simulink model "FuzzyPID_modle"  (R2024b)
settings: Solver=ode4  StartTime=0.0  StopTime=100  FixedStep=0.5  RelTol=1e-3
undefined symbols (not defined in the file): DiscIntNeverNeededParam
libraries: fuzblock x2, slpidlib x1
settings Model: Creator=33242  LastModifiedBy=33242

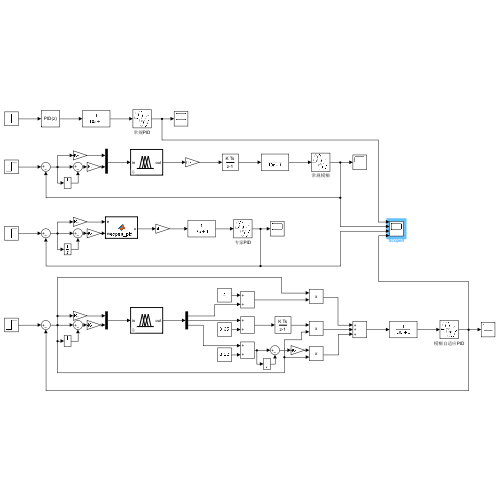
[thumbnail: Simulink's stored preview of the top-level diagram]
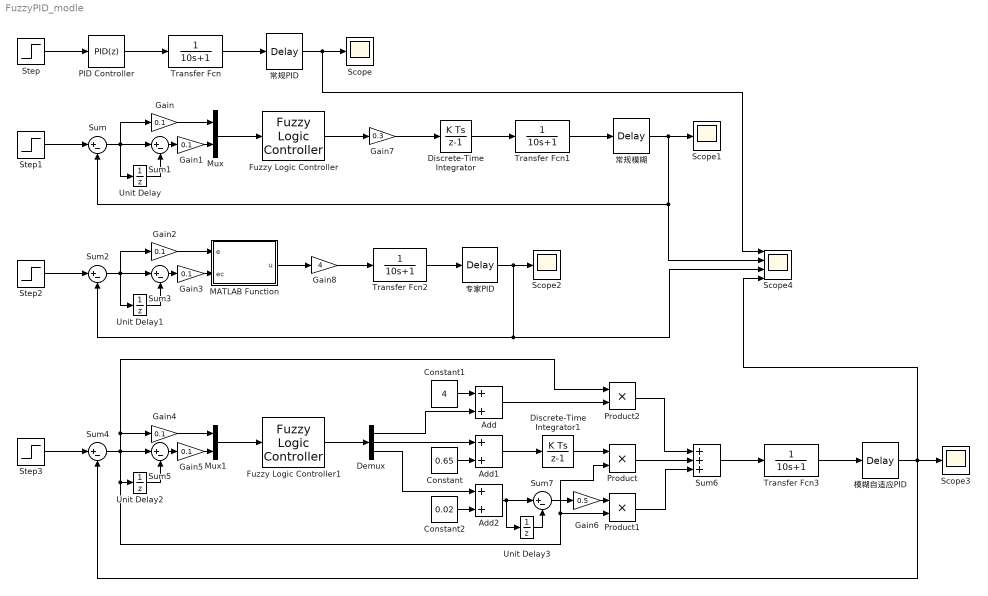
== system FuzzyPID_modle ==
  Add : Sum
  Add1 : Sum
  Add2 : Sum
  Constant : Constant  Value=0.65
  Constant1 : Constant  Value=4
  Constant2 : Constant  Value=0.02
  Demux : Demux  Outputs=3
  Discrete-Time Integrator : DiscreteIntegrator  SampleTime=0.5  ICPrevOutput=DiscIntNeverNeededParam  ICPrevScaledInput=DiscIntNeverNeededParam
  Discrete-Time Integrator1 : DiscreteIntegrator  SampleTime=0.5  ICPrevOutput=DiscIntNeverNeededParam  ICPrevScaledInput=DiscIntNeverNeededParam
  Fuzzy Logic Controller : fuzblock/Fuzzy Logic  Controller  FIS=fuzzyPID  OutputSampleNumber=101  DataType=double  FuzzifiedInputs=off  RuleFiringStrengths=off  RuleOutputs=off  AggregatedOutputs=off  SimulateUsing=Interpreted execution  OutOfRangeInputValueMessage=warning  NoRuleFiredMessage=warning  EmptyOutputFuzzySetMessage=warning
  Fuzzy Logic Controller1 : fuzblock/Fuzzy Logic  Controller  FIS=FUZZYpid  OutputSampleNumber=101  DataType=double  FuzzifiedInputs=off  RuleFiringStrengths=off  RuleOutputs=off  AggregatedOutputs=off  SimulateUsing=Interpreted execution  OutOfRangeInputValueMessage=warning  NoRuleFiredMessage=warning  EmptyOutputFuzzySetMessage=warning
  Gain{,1..5} (6 alike) : Gain  Gain=0.1
  Gain6 : Gain  Gain=0.5
  Gain7 : Gain  Gain=0.3
  Gain8 : Gain  Gain=4
  MATLAB Function : MATLAB Function  TreatAsAtomicUnit=on
  Mux : Mux  Inputs=2
  Mux1 : Mux  Inputs=2
  PID Controller : slpidlib/PID Controller  Controller=PID  Form=Parallel  TimeDomain=Discrete-time  UseExternalTs=off  SampleTime=0.5  IntegratorMethod=Forward Euler  FilterMethod=Forward Euler  ControllerParametersSource=internal  P=1  I=0  UseKiTs=off  D=0  UseExternalDerivativeSource=off  N=100  UseFilter=on  TunerSelectOption=Transfer Function Based (PID Tuner App)  InitialConditionSource=internal  InitialConditionForIntegrator=0  InitialConditionForFilter=0  DifferentiatorICPrevScaledInput=0  ExternalReset=none  TrackingMode=off  Kt=1  LimitOutput=off  SatLimitsSource=internal  UpperSaturationLimit=inf  LowerSaturationLimit=-inf  LinearizeAsGain=on  AntiWindupMode=none  Kb=1  LimitIntegrator=off  UpperIntegratorSaturationLimit=inf  LowerIntegratorSaturationLimit=-inf  POutMin=[]  POutMax=[]  IOutMin=[]  IOutMax=[]  DOutMin=[]  DOutMax=[]  NOutMin=[]  NOutMax=[]  SumOutMin=[]  SumOutMax=[]  SaturationOutMin=[]  SaturationOutMax=[]  PParamMin=[]  PParamMax=[]  IParamMin=[]  IParamMax=[]  DParamMin=[]  DParamMax=[]  NParamMin=[]  NParamMax=[]  KbParamMin=[]  KbParamMax=[]  KtParamMin=[]  KtParamMax=[]  KbOutMin=[]  KbOutMax=[]  KtOutMin=[]  KtOutMax=[]  IntegratorOutMin=[]  IntegratorOutMax=[]  FilterOutMin=[]  FilterOutMax=[]  SumI1OutMin=[]  SumI1OutMax=[]  SumI2OutMin=[]  SumI2OutMax=[]  SumI3OutMin=[]  SumI3OutMax=[]  SumI4OutMin=[]  SumI4OutMax=[]  SumDOutMin=[]  SumDOutMax=[]  DifferentiatorOutMin=[]  DifferentiatorOutMax=[]  FilterDiffOutCoefMin=[]  FilterDiffOutCoefMax=[]  ReciprocalOutMin=[]  ReciprocalOutMax=[]  SumDenOutMin=[]  SumDenOutMax=[]  SumNumOutMin=[]  SumNumOutMax=[]  DivideOutMin=[]  DivideOutMax=[]  UdiffTsProdOutMin=[]  UdiffTsProdOutMax=[]  NTsProdOutMin=[]  NTsProdOutMax=[]  UintegralTsProdOutMin=[]  UintegralTsProdOutMax=[]  UngainTsProdOutMin=[]  UngainTsProdOutMax=[]  ClampingZeroOutDataTypeStr=Inherit: Inherit via back propagation  ClampingZeroOutMin=[]  ClampingZeroOutMax=[]  FilterDenConstantOutDataTypeStr=Inherit: Inherit via back propagation  FilterDenConstantOutMin=[]  FilterDenConstantOutMax=[]  PCopyOutDataTypeStr=Inherit: Inherit via back propagation  PCopyOutMin=[]  PCopyOutMax=[]  NCopyOutDataTypeStr=Inherit: Inherit via back propagation  NCopyOutMin=[]  NCopyOutMax=[]  IntegratorContinuousStateAttributes=''  IntegratorStateMustResolveToSignalObject=off  IntegratorRTWStateStorageClass=Auto  FilterContinuousStateAttributes=''  FilterStateMustResolveToSignalObject=off  FilterRTWStateStorageClass=Auto  ParallelPVariant=InternalParameters  IdealPVariant=Disabled  IVariant=InternalParameters  DVariant=InternalParameters  IntegratorVariant=Discrete  SatVariant=Disabled  AWVariant=Passthrough  PCopyVariant=Disabled  TRVariant=Disabled  FdbkBlocksVariant=Forward  IdealPFdbkVariant=Disabled  SatFdbkVariant=Disabled  DerivativeFilterVariant=ForwardEulerFilter  NVariant=InternalParameters  NCopyVariant=Disabled  FilterICVariant=InternalICsFilter  IntegratorICVariant=InternalICs  ExternalResetVariant=Disabled  TRSumVariant=Passthrough  SumFdbkVariant=Disabled  SumVariant=Sum_PID  TsampFilterVariant=InternalTs  TsampNgainVariant=Passthrough  TsampIntegralVariant=Disabled_SignalSpec  ExternalSaturationOutDataTypeStr=Inherit: Same as second input  DerivativeSourceVariant=ErrorSignal  PreIntVariant=InternalPreInt
  Product : Product
  Product1 : Product
  Product2 : Product
  Scope{,1..3} (4 alike) : Scope
  Scope4 : Scope  NumInputPorts=4
  Step{,1..3} (4 alike) : Step  Time=0  After=30  SampleTime=0
  Sum{,1..5,7} (7 alike) : Sum  Inputs=|+-
  Sum6 : Sum  Inputs=+++
  Transfer Fcn{,1..3} (4 alike) : TransferFcn  Denominator=[10 1]
  Unit Delay{,1..3} (4 alike) : UnitDelay  SampleTime=0.5  HasFrameUpgradeWarning=on
  专家PID : TransportDelay  DelayTime=0.5
  常规PID : TransportDelay  DelayTime=0.5
  常规模糊 : TransportDelay  DelayTime=0.5
  模糊自适应PID : TransportDelay  DelayTime=0.5
  wires:
  Transfer Fcn/1 -> 常规PID/1
  常规PID/1 -> Scope/1, Scope4/1
  Sum/1 -> Gain/1, Unit Delay/1, Sum1/1
  Unit Delay/1 -> Sum1/2
  Mux/1 -> Fuzzy Logic Controller/1
  Fuzzy Logic Controller/1 -> Gain7/1
  Discrete-Time Integrator/1 -> Transfer Fcn1/1
  Transfer Fcn1/1 -> 常规模糊/1
  常规模糊/1 -> Sum/2, Scope4/2, Scope1/1
  Step1/1 -> Sum/1
  PID Controller/1 -> Transfer Fcn/1
  Step/1 -> PID Controller/1
  Step2/1 -> Sum2/1
  Unit Delay1/1 -> Sum3/2
  Sum2/1 -> Gain2/1, Sum3/1, Unit Delay1/1
  MATLAB Function/1(u) -> Gain8/1
  Transfer Fcn2/1 -> 专家PID/1
  专家PID/1 -> Scope2/1, Scope4/3, Sum2/2
  Step3/1 -> Sum4/1
  Unit Delay2/1 -> Sum5/2
  Sum4/1 -> Sum5/1, Product1/2, Product/2, Unit Delay2/1, Product2/1, Gain4/1
  Mux1/1 -> Fuzzy Logic Controller1/1
  Fuzzy Logic Controller1/1 -> Demux/1
  Constant/1 -> Add1/2
  Constant1/1 -> Add/1
  Constant2/1 -> Add2/2
  Add/1 -> Product2/2
  Add1/1 -> Discrete-Time Integrator1/1
  Product/1 -> Sum6/2
  Product2/1 -> Sum6/1
  Product1/1 -> Sum6/3
  模糊自适应PID/1 -> Sum4/2, Scope4/4, Scope3/1
  Transfer Fcn3/1 -> 模糊自适应PID/1
  Sum6/1 -> Transfer Fcn3/1
  Discrete-Time Integrator1/1 -> Product/1
  Gain/1 -> Mux/1
  Sum1/1 -> Gain1/1
  Gain1/1 -> Mux/2
  Gain2/1 -> MATLAB Function/1(e)
  Sum3/1 -> Gain3/1
  Gain3/1 -> MATLAB Function/2(ec)
  Gain4/1 -> Mux1/1
  Sum5/1 -> Gain5/1
  Gain5/1 -> Mux1/2
  Add2/1 -> Unit Delay3/1, Sum7/1
  Gain6/1 -> Product1/1
  Unit Delay3/1 -> Sum7/2
  Sum7/1 -> Gain6/1
  Gain7/1 -> Discrete-Time Integrator/1
  Gain8/1 -> Transfer Fcn2/1
  Demux/1 -> Add/2
  Demux/2 -> Add1/1
  Demux/3 -> Add2/1

== matlab function FuzzyPID_modle/MATLAB Function ==
  settings: updateMethod=DISCRETE  sampleTime=0.5
  data: e input; u output; ec input
function u = expert_pid(e, ec)
    % 初始化持久变量（用于保存上一时刻的误差和积分项）
    persistent e_1 e_2 u_k
    if isempty(e_1)
        e_1 = 0; e_2 = 0; u_k = 0;
    end
    
    % 设定基础参数（需根据常规PID整定结果填入）
    kp = 2.0; ki = 0.5; kd = 0.1; 
    
    % 设定专家规则的阈值
    M1 = 15; % 最大误差界限
    M2 = 5;  % 中等误差界限
    
    % --- 专家规则判断开始 ---
    if abs(e) > M1
        % 规则1：误差极大，实施开环 Bang-Bang 控制，全速赶往目标
        u_k = u_k + kp * 2.0 * sign(e); % 强输出
        
    elseif e * ec > 0 || ec == 0
        % 规则2：误差在增大，或者误差没有减小趋势，需增强控制作用
        if abs(e) > M2
            u_k = u_k + kp*(e-e_1) + ki*e + kd*(e - 2*e_1 + e_2); % 较强的PID增量
        else
            u_k = u_k + 0.8*kp*(e-e_1) + ki*e + kd*(e - 2*e_1 + e_2); % 较弱的PID增量
        end
        
    elseif e * ec < 0 && e * e_1 > 0
        % 规则3：误差在减小，保持现有控制即可
        u_k = u_k; 
        
    elseif abs(e) < 0.5
        % 规则4：误差极小，加入强积分作用消除静差
        u_k = u_k + kp*(e-e_1) + 1.5*ki*e; 
    else
        % 规则5：其他情况，采用常规离散增量PID
        u_k = u_k + kp*(e-e_1) + ki*e + kd*(e - 2*e_1 + e_2);
    end
    
    % 更新历史状态
    e_2 = e_1;
    e_1 = e;
    u = u_k;
end
